simulink model "Buck_28V_12V_Analysis"  (R2023a)
settings: Solver=ode23t  StartTime=0.0  StopTime=0.05  MaxStep=1e-6  RelTol=1e-3
undefined symbols (not defined in the file): Rload
libraries: ee_lib x34, nesl_utility x33, fl_lib x26, simulink x24, slpidlib x4, simulink_extras x3
(part 1 of 2)
settings Model: Creator=MEHMET  LastModifiedBy=MEHMET

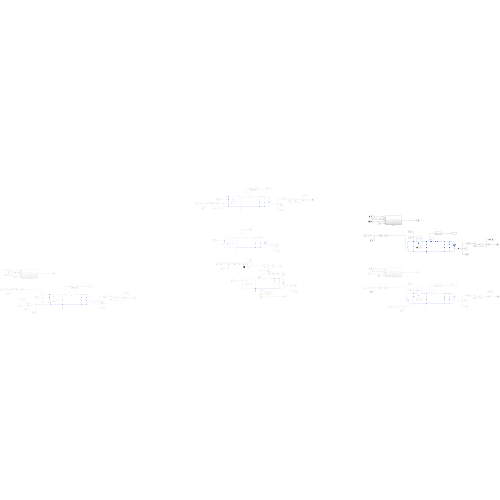
[thumbnail: Simulink's stored preview of the top-level diagram]
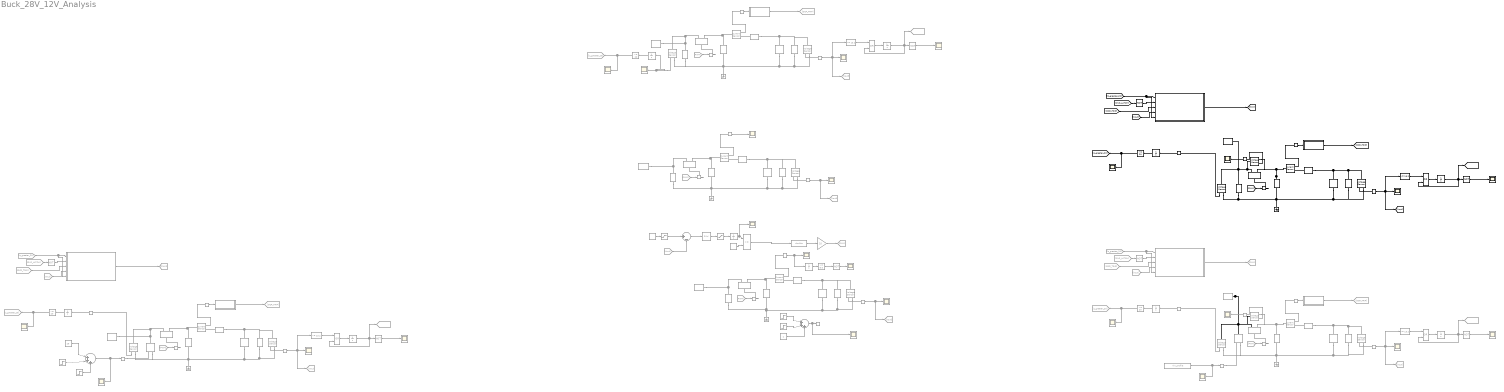
== system Buck_28V_12V_Analysis ==
  Capacitor{,1..3} (4 alike) : ee_lib/Passive/Capacitor  Commented=on  cap_option=ee.enum.passive.capacitor.capOption.const  c=220 uF  Cvec=[1e-05, 1e-06] F  Vvec=[0, 10] V  CV_table_symmetry=ee.enum.passive.capacitor.tableSymmetry.yes  f_vec=[1, 10] kHz  DFext_vec=[.8, 1.2]  enable_C_tol=ee.enum.toleranceApplication.none  averaging_period=0 s  C_tol=5  tol_distribution=ee.enum.toleranceDistribution.uniform  nSigma=4  r=1e-6 Ohm  g=0 1/Ohm  enable_operating_limits=ee.enum.enable.no  enable_faults=ee.enum.enable.no  fault_action=simscape.enum.assert.action.none  Cscale_faulted=100  R_faulted=1e-3 Ohm  G_faulted=0 1/Ohm  tau_fault=1e-3 s  fault_trigger=ee.enum.faults.faultTrigger.temporal  t_fault=1 s  max_permissible_voltage_range=[-100, 100] V  t_fail_on_voltage=1 s  operating_limit_action=ee.enum.passive.reportOpLim.warn  max_working_voltage_range=[-25, 25] V  power_rating=1 W  i_specify=off  i_priority=None  i=0 A  i_nominal_specify=off  i_nominal_unit=A  i_nominal_value=1  v_specify=off  v_priority=None  v=0 V  v_nominal_specify=off  v_nominal_unit=V  v_nominal_value=1  vc_specify=off  vc_priority=High  vc=0 V  vc_nominal_specify=off  vc_nominal_unit=V  vc_nominal_value=1
  Capacitor4 : ee_lib/Passive/Capacitor  cap_option=ee.enum.passive.capacitor.capOption.const  c=220 uF  Cvec=[1e-05, 1e-06] F  Vvec=[0, 10] V  CV_table_symmetry=ee.enum.passive.capacitor.tableSymmetry.yes  f_vec=[1, 10] kHz  DFext_vec=[.8, 1.2]  enable_C_tol=ee.enum.toleranceApplication.none  averaging_period=0 s  C_tol=5  tol_distribution=ee.enum.toleranceDistribution.uniform  nSigma=4  r=1e-6 Ohm  g=0 1/Ohm  enable_operating_limits=ee.enum.enable.no  enable_faults=ee.enum.enable.no  fault_action=simscape.enum.assert.action.none  Cscale_faulted=100  R_faulted=1e-3 Ohm  G_faulted=0 1/Ohm  tau_fault=1e-3 s  fault_trigger=ee.enum.faults.faultTrigger.temporal  t_fault=1 s  max_permissible_voltage_range=[-100, 100] V  t_fail_on_voltage=1 s  operating_limit_action=ee.enum.passive.reportOpLim.warn  max_working_voltage_range=[-25, 25] V  power_rating=1 W  i_specify=off  i_priority=None  i=0 A  i_nominal_specify=off  i_nominal_unit=A  i_nominal_value=1  v_specify=off  v_priority=None  v=0 V  v_nominal_specify=off  v_nominal_unit=V  v_nominal_value=1  vc_specify=off  vc_priority=High  vc=0 V  vc_nominal_specify=off  vc_nominal_unit=V  vc_nominal_value=1
  Capacitor5 : ee_lib/Passive/Capacitor  Commented=on  cap_option=ee.enum.passive.capacitor.capOption.const  c=C_test F  Cvec=[1e-05, 1e-06] F  Vvec=[0, 10] V  CV_table_symmetry=ee.enum.passive.capacitor.tableSymmetry.yes  f_vec=[1, 10] kHz  DFext_vec=[.8, 1.2]  enable_C_tol=ee.enum.toleranceApplication.none  averaging_period=0 s  C_tol=5  tol_distribution=ee.enum.toleranceDistribution.uniform  nSigma=4  r=ESR_test Ohm  g=0 1/Ohm  enable_operating_limits=ee.enum.enable.no  enable_faults=ee.enum.enable.no  fault_action=simscape.enum.assert.action.none  Cscale_faulted=100  R_faulted=1e-3 Ohm  G_faulted=0 1/Ohm  tau_fault=1e-3 s  fault_trigger=ee.enum.faults.faultTrigger.temporal  t_fault=1 s  max_permissible_voltage_range=[-100, 100] V  t_fail_on_voltage=1 s  operating_limit_action=ee.enum.passive.reportOpLim.warn  max_working_voltage_range=[-25, 25] V  power_rating=1 W  i_specify=off  i_priority=None  i=0 A  i_nominal_specify=off  i_nominal_unit=A  i_nominal_value=1  v_specify=off  v_priority=None  v=0 V  v_nominal_specify=off  v_nominal_unit=V  v_nominal_value=1  vc_specify=off  vc_priority=High  vc=0 V  vc_nominal_specify=off  vc_nominal_unit=V  vc_nominal_value=1
  Compare : Scope  Commented=on
  Compare To Constant : simulink/Logic and Bit Operations/Compare To Constant  Commented=on  relop=>=  const=6.0  OutDataTypeStr=boolean  ZeroCross=off
  Compare To Constant1 : simulink/Logic and Bit Operations/Compare To Constant  Commented=on  relop=>=  const=13.2  OutDataTypeStr=boolean  ZeroCross=off
  Compare To Constant2 : simulink/Logic and Bit Operations/Compare To Constant  Commented=on  relop=>=  const=20  OutDataTypeStr=boolean  ZeroCross=off
  Compare To Constant3 : simulink/Logic and Bit Operations/Compare To Constant  Commented=on  relop=>=  const=13.2  OutDataTypeStr=boolean  ZeroCross=off
  Compare To Constant4 : simulink/Logic and Bit Operations/Compare To Constant  Commented=on  relop=>=  const=20  OutDataTypeStr=boolean  ZeroCross=off
  Compare To Constant5 : simulink/Logic and Bit Operations/Compare To Constant  relop=>=  const=13.2  OutDataTypeStr=boolean  ZeroCross=off
  Compare To Constant6 : simulink/Logic and Bit Operations/Compare To Constant  relop=>=  const=20  OutDataTypeStr=boolean  ZeroCross=off
  Compare To Constant7 : simulink/Logic and Bit Operations/Compare To Constant  Commented=on  relop=>=  const=13.2  OutDataTypeStr=boolean  ZeroCross=off
  Compare To Constant8 : simulink/Logic and Bit Operations/Compare To Constant  Commented=on  relop=>=  const=20  OutDataTypeStr=boolean  ZeroCross=off
  Constant : Constant  Commented=on  Value=28
  Constant1 : Constant  Commented=on
  Controlled Voltage Source : fl_lib/Electrical/Electrical Sources/Controlled Voltage Source  Commented=on
  Controlled Voltage Source1 : fl_lib/Electrical/Electrical Sources/Controlled Voltage Source  Commented=on
  Current Sensor{,1..3,5} (5 alike) : fl_lib/Electrical/Electrical Sensors/Current Sensor  Commented=on
  Current Sensor4 : fl_lib/Electrical/Electrical Sensors/Current Sensor
  Current_Scope : Scope  Commented=on
  Current_Scope1 : Scope  Commented=on
  Current_is_greater_6A : Subsystem  Commented=on
  Current_is_greater_6A1 : Subsystem  Commented=on
  Current_is_greater_6A2 : Subsystem
  Current_is_greater_6A3 : Subsystem  Commented=on
  DC Voltage Source : ee_lib/Additional Components/SPICE Sources/DC Voltage Source  Commented=on  DC=28 V
  DC Voltage Source1 : ee_lib/Additional Components/SPICE Sources/DC Voltage Source  Commented=on  DC=Vin V
  DC Voltage Source2 : ee_lib/Additional Components/SPICE Sources/DC Voltage Source  Commented=on  DC=Vin V
  DC Voltage Source3 : ee_lib/Additional Components/SPICE Sources/DC Voltage Source  DC=28 V
  Data Type Conversion : DataTypeConversion  Commented=on  OutDataTypeStr=double  SaturateOnIntegerOverflow=off  RndMeth=Floor
  Diode{,1..3} (4 alike) : ee_lib/Semiconductors & Converters/Diode  Commented=on  ModelType=ee.enum.diode.modelType.pwl  TableType=ee.enum.diode.tableType.IfMat  IfMat=[.07, .12, .19, 1.75, 4.24, 7.32, 11.2; .16, .3, .72, 2.14, 5.02, 8.35, 13.12] A  VfMat=[.9, 1.15, 1.25, 1.5, 1.75, 2.17, 2.6, 2.85; .58, .68, .75, 1.1, 1.38, 1.77, 2.27, 2.7] V  TjVec=[25, 125] degC  VfVec=[.5, .7, .9, 1.3, 1.7, 2.1, 2.5] V  IfVec=[.1, .2, .5, 1, 2, 4, 7, 10] A  Vf=0.6 V  Ron=0.3 Ohm  Goff=1e-8 S  prmExp=ee.enum.diode.expParam.useTwo  I12=[.0137, .545] A  V12=[.6, .7] V  RS=0 Ohm  Tmeas=25 degC  IS=1e-12 A  ec=1  I1=0.0137 A  V1=0.6 V  N_series=1  N_parallel=1  Rz=0.3 Ohm  BV=inf V  C_param=ee.enum.diode.capParam.fixed  CJ=0 pF  CJ0=5 pF  Vvec=[.1, 10, 100] V  Cvec=[3.5, 1, .4] pF  VJ=1 V  Mgrad=0.5  FC=0.5  Q_param=ee.enum.diode.recoveryParam.off  iRM=-7.15 A  iF=4 A  didt=-750 A/us  trr_factor=3  trr=115 ns  Qrr=150 nA*s  Vr=-600 V  Ls=150 nH  Erec=0.03 J  TT=50 ns  tau=100 ns  T_param=ee.enum.diode.temperatureParam.off  Tdevice=25 degC  I1_T2=0.245 A  V1_T2=0.5 V  IS_T2=1.25e-7 A  Tmeas2=125 degC  XTI_param=ee.enum.diode.xtiParam.pn  XTI=3  EG_param=ee.enum.diode.egapParam.material_si  EG=1.11 eV  dBVdT=0 V/K  enable_faults=simscape.enum.onoff.off  fault_action=simscape.enum.assert.action.none  fault_types=ee.enum.diode.faults.open  tau_fault=1e-3 s  IfMat_faulted=[.07, .12, .19, 1.75, 4.24, 7.32, 11.2; .16, .3, .72, 2.14, 4.02, 6.35, 9.12] A  VfMat_faulted=[.9, 1.15, 1.25, 1.5, 1.75, 2.17, 2.6, 2.85; .58, .68, .75, 1.1, 1.38, 1.77, 2.27, 2.7] V  VfVec_faulted=[.5, .7, .9, 1.3, 1.7, 2.1, 2.5] V  IfVec_faulted=[.1, .2, .5, 1, 2, 4, 7, 10] A  Ropen_faulted=1000 Ohm  Gshort_faulted=1000 1/Ohm  Vf_faulted=0.6 V  Ron_faulted=0.3 Ohm  Goff_faulted=1e-8 S  I12_faulted=[.0137, .545] A  V12_faulted=[.6, .7] V  IS_faulted=1e-12 A  ec_faulted=1  I1_faulted=0.0137 A  V1_faulted=0.6 V  RS_faulted=0 Ohm  Rz_faulted=0.3 Ohm  BV_faulted=inf V  Cscale_faulted=100  fault_trigger=ee.enum.faults.faultTrigger.temporal  t_fault=inf s  max_permissible_voltage=inf V  n_fail_on_voltage=1  max_permissible_current=inf A  t_fail_on_current=1 s  max_permissible_dVdt=inf V/s  enable_fault_input=simscape.enum.onoff.off  i_specify=off  i_priority=None  i=0 A  i_nominal_specify=off  i_nominal_unit=A  i_nominal_value=1  v_specify=off  v_priority=None  v=0 V  v_nominal_specify=off  v_nominal_unit=V  v_nominal_value=1  v_capacitor_specify=off  v_capacitor_priority=None  v_capacitor=0 V  v_capacitor_nominal_specify=off  v_capacitor_nominal_unit=V  v_capacitor_nominal_value=1  i_diode_specify=off  i_diode_priority=None  i_diode=0 A  i_diode_nominal_specify=off  i_diode_nominal_unit=A  i_diode_nominal_value=1  v_diode_specify=off  v_diode_priority=None  v_diode=0 V  v_diode_nominal_specify=off  v_diode_nominal_unit=V  v_diode_nominal_value=1  i_capacitor_specify=off  i_capacitor_priority=None  i_capacitor=0 A  i_capacitor_nominal_specify=off  i_capacitor_nominal_unit=A  i_capacitor_nominal_value=1  power_dissipated_specify=off  power_dissipated_priority=None  power_dissipated=0 W  power_dissipated_nominal_specify=off  power_dissipated_nominal_unit=W  power_dissipated_nominal_value=1  fidelity_level=ee.enum.diode.fidelity.includeChargeDyn  rec_loss_model=ee.enum.diode.reverseRecoveryModel.fixed  ErecVal=0 J  ErecMat=zeros(2, 3) J  TjrecVec=[298.15, 398.15] K  IfrecVec=[.1, 1, 10] A  VrecVal=10 V  tFilter=1 / 1000 / 100 s  max_permissible_temperature=inf K  t_fail_on_temperature=1 s  thermal_network_parameterization=ee.enum.thermalNetworkTopology.junctionCase  Rth=[0, 10] K/W  Rth_Cauer=[1, 3, 10] K/W  Rth_Foster=[4, 6] K/W  thermal_mass_parameterization=ee.enum.thermalNetwork.timeconstant  thermal_mass=[0, 1] J/K  thermal_mass_Cauer=[.1, .3, 1] J/K  thermal_mass_Foster=[1.5, 3] J/K  thermal_time_constant=[0, 10] s  thermal_time_constant_Cauer=[1, 3, 10] s  thermal_time_constant_Foster=[6, 18] s  thermal_mass_initial_temperatures=[25, 25] degC  thermal_mass_initial_temperatures_Cauer=[25, 25, 25] degC  junction_thermal_mass=0.01 J/K  Tvec_initial_Foster=[25, 25, 25, 25] degC  no_thermal_network=0  junction_temperature_specify=off  junction_temperature_priority=None  junction_temperature=25 degC  junction_temperature_nominal_specify=off  junction_temperature_nominal_unit=degC  junction_temperature_nominal_value=1
  Diode4 : ee_lib/Semiconductors & Converters/Diode  ModelType=ee.enum.diode.modelType.pwl  TableType=ee.enum.diode.tableType.IfMat  IfMat=[.07, .12, .19, 1.75, 4.24, 7.32, 11.2; .16, .3, .72, 2.14, 5.02, 8.35, 13.12] A  VfMat=[.9, 1.15, 1.25, 1.5, 1.75, 2.17, 2.6, 2.85; .58, .68, .75, 1.1, 1.38, 1.77, 2.27, 2.7] V  TjVec=[25, 125] degC  VfVec=[.5, .7, .9, 1.3, 1.7, 2.1, 2.5] V  IfVec=[.1, .2, .5, 1, 2, 4, 7, 10] A  Vf=0.6 V  Ron=0.3 Ohm  Goff=1e-8 S  prmExp=ee.enum.diode.expParam.useTwo  I12=[.0137, .545] A  V12=[.6, .7] V  RS=0 Ohm  Tmeas=25 degC  IS=1e-12 A  ec=1  I1=0.0137 A  V1=0.6 V  N_series=1  N_parallel=1  Rz=0.3 Ohm  BV=inf V  C_param=ee.enum.diode.capParam.fixed  CJ=0 pF  CJ0=5 pF  Vvec=[.1, 10, 100] V  Cvec=[3.5, 1, .4] pF  VJ=1 V  Mgrad=0.5  FC=0.5  Q_param=ee.enum.diode.recoveryParam.off  iRM=-7.15 A  iF=4 A  didt=-750 A/us  trr_factor=3  trr=115 ns  Qrr=150 nA*s  Vr=-600 V  Ls=150 nH  Erec=0.03 J  TT=50 ns  tau=100 ns  T_param=ee.enum.diode.temperatureParam.off  Tdevice=25 degC  I1_T2=0.245 A  V1_T2=0.5 V  IS_T2=1.25e-7 A  Tmeas2=125 degC  XTI_param=ee.enum.diode.xtiParam.pn  XTI=3  EG_param=ee.enum.diode.egapParam.material_si  EG=1.11 eV  dBVdT=0 V/K  enable_faults=simscape.enum.onoff.off  fault_action=simscape.enum.assert.action.none  fault_types=ee.enum.diode.faults.open  tau_fault=1e-3 s  IfMat_faulted=[.07, .12, .19, 1.75, 4.24, 7.32, 11.2; .16, .3, .72, 2.14, 4.02, 6.35, 9.12] A  VfMat_faulted=[.9, 1.15, 1.25, 1.5, 1.75, 2.17, 2.6, 2.85; .58, .68, .75, 1.1, 1.38, 1.77, 2.27, 2.7] V  VfVec_faulted=[.5, .7, .9, 1.3, 1.7, 2.1, 2.5] V  IfVec_faulted=[.1, .2, .5, 1, 2, 4, 7, 10] A  Ropen_faulted=1000 Ohm  Gshort_faulted=1000 1/Ohm  Vf_faulted=0.6 V  Ron_faulted=0.3 Ohm  Goff_faulted=1e-8 S  I12_faulted=[.0137, .545] A  V12_faulted=[.6, .7] V  IS_faulted=1e-12 A  ec_faulted=1  I1_faulted=0.0137 A  V1_faulted=0.6 V  RS_faulted=0 Ohm  Rz_faulted=0.3 Ohm  BV_faulted=inf V  Cscale_faulted=100  fault_trigger=ee.enum.faults.faultTrigger.temporal  t_fault=inf s  max_permissible_voltage=inf V  n_fail_on_voltage=1  max_permissible_current=inf A  t_fail_on_current=1 s  max_permissible_dVdt=inf V/s  enable_fault_input=simscape.enum.onoff.off  i_specify=off  i_priority=None  i=0 A  i_nominal_specify=off  i_nominal_unit=A  i_nominal_value=1  v_specify=off  v_priority=None  v=0 V  v_nominal_specify=off  v_nominal_unit=V  v_nominal_value=1  v_capacitor_specify=off  v_capacitor_priority=None  v_capacitor=0 V  v_capacitor_nominal_specify=off  v_capacitor_nominal_unit=V  v_capacitor_nominal_value=1  i_diode_specify=off  i_diode_priority=None  i_diode=0 A  i_diode_nominal_specify=off  i_diode_nominal_unit=A  i_diode_nominal_value=1  v_diode_specify=off  v_diode_priority=None  v_diode=0 V  v_diode_nominal_specify=off  v_diode_nominal_unit=V  v_diode_nominal_value=1  i_capacitor_specify=off  i_capacitor_priority=None  i_capacitor=0 A  i_capacitor_nominal_specify=off  i_capacitor_nominal_unit=A  i_capacitor_nominal_value=1  power_dissipated_specify=off  power_dissipated_priority=None  power_dissipated=0 W  power_dissipated_nominal_specify=off  power_dissipated_nominal_unit=W  power_dissipated_nominal_value=1  fidelity_level=ee.enum.diode.fidelity.includeChargeDyn  rec_loss_model=ee.enum.diode.reverseRecoveryModel.fixed  ErecVal=0 J  ErecMat=zeros(2, 3) J  TjrecVec=[298.15, 398.15] K  IfrecVec=[.1, 1, 10] A  VrecVal=10 V  tFilter=1 / 1000 / 100 s  max_permissible_temperature=inf K  t_fail_on_temperature=1 s  thermal_network_parameterization=ee.enum.thermalNetworkTopology.junctionCase  Rth=[0, 10] K/W  Rth_Cauer=[1, 3, 10] K/W  Rth_Foster=[4, 6] K/W  thermal_mass_parameterization=ee.enum.thermalNetwork.timeconstant  thermal_mass=[0, 1] J/K  thermal_mass_Cauer=[.1, .3, 1] J/K  thermal_mass_Foster=[1.5, 3] J/K  thermal_time_constant=[0, 10] s  thermal_time_constant_Cauer=[1, 3, 10] s  thermal_time_constant_Foster=[6, 18] s  thermal_mass_initial_temperatures=[25, 25] degC  thermal_mass_initial_temperatures_Cauer=[25, 25, 25] degC  junction_thermal_mass=0.01 J/K  Tvec_initial_Foster=[25, 25, 25, 25] degC  no_thermal_network=0  junction_temperature_specify=off  junction_temperature_priority=None  junction_temperature=25 degC  junction_temperature_nominal_specify=off  junction_temperature_nominal_unit=degC  junction_temperature_nominal_value=1
  Diode5 : ee_lib/Semiconductors & Converters/Diode  Commented=on  ModelType=ee.enum.diode.modelType.pwl  TableType=ee.enum.diode.tableType.IfMat  IfMat=[.07, .12, .19, 1.75, 4.24, 7.32, 11.2; .16, .3, .72, 2.14, 5.02, 8.35, 13.12] A  VfMat=[.9, 1.15, 1.25, 1.5, 1.75, 2.17, 2.6, 2.85; .58, .68, .75, 1.1, 1.38, 1.77, 2.27, 2.7] V  TjVec=[25, 125] degC  VfVec=[.5, .7, .9, 1.3, 1.7, 2.1, 2.5] V  IfVec=[.1, .2, .5, 1, 2, 4, 7, 10] A  Vf=0.6 V  Ron=0.01 Ohm  Goff=1e-8 S  prmExp=ee.enum.diode.expParam.useTwo  I12=[.0137, .545] A  V12=[.6, .7] V  RS=0 Ohm  Tmeas=25 degC  IS=1e-12 A  ec=1  I1=0.0137 A  V1=0.6 V  N_series=1  N_parallel=1  Rz=0.3 Ohm  BV=inf V  C_param=ee.enum.diode.capParam.fixed  CJ=0 pF  CJ0=5 pF  Vvec=[.1, 10, 100] V  Cvec=[3.5, 1, .4] pF  VJ=1 V  Mgrad=0.5  FC=0.5  Q_param=ee.enum.diode.recoveryParam.off  iRM=-7.15 A  iF=4 A  didt=-750 A/us  trr_factor=3  trr=115 ns  Qrr=150 nA*s  Vr=-600 V  Ls=150 nH  Erec=0.03 J  TT=50 ns  tau=100 ns  T_param=ee.enum.diode.temperatureParam.off  Tdevice=25 degC  I1_T2=0.245 A  V1_T2=0.5 V  IS_T2=1.25e-7 A  Tmeas2=125 degC  XTI_param=ee.enum.diode.xtiParam.pn  XTI=3  EG_param=ee.enum.diode.egapParam.material_si  EG=1.11 eV  dBVdT=0 V/K  enable_faults=simscape.enum.onoff.off  fault_action=simscape.enum.assert.action.none  fault_types=ee.enum.diode.faults.open  tau_fault=1e-3 s  IfMat_faulted=[.07, .12, .19, 1.75, 4.24, 7.32, 11.2; .16, .3, .72, 2.14, 4.02, 6.35, 9.12] A  VfMat_faulted=[.9, 1.15, 1.25, 1.5, 1.75, 2.17, 2.6, 2.85; .58, .68, .75, 1.1, 1.38, 1.77, 2.27, 2.7] V  VfVec_faulted=[.5, .7, .9, 1.3, 1.7, 2.1, 2.5] V  IfVec_faulted=[.1, .2, .5, 1, 2, 4, 7, 10] A  Ropen_faulted=1000 Ohm  Gshort_faulted=1000 1/Ohm  Vf_faulted=0.6 V  Ron_faulted=0.3 Ohm  Goff_faulted=1e-8 S  I12_faulted=[.0137, .545] A  V12_faulted=[.6, .7] V  IS_faulted=1e-12 A  ec_faulted=1  I1_faulted=0.0137 A  V1_faulted=0.6 V  RS_faulted=0 Ohm  Rz_faulted=0.3 Ohm  BV_faulted=inf V  Cscale_faulted=100  fault_trigger=ee.enum.faults.faultTrigger.temporal  t_fault=inf s  max_permissible_voltage=inf V  n_fail_on_voltage=1  max_permissible_current=inf A  t_fail_on_current=1 s  max_permissible_dVdt=inf V/s  enable_fault_input=simscape.enum.onoff.off  i_specify=off  i_priority=None  i=0 A  i_nominal_specify=off  i_nominal_unit=A  i_nominal_value=1  v_specify=off  v_priority=None  v=0 V  v_nominal_specify=off  v_nominal_unit=V  v_nominal_value=1  v_capacitor_specify=off  v_capacitor_priority=None  v_capacitor=0 V  v_capacitor_nominal_specify=off  v_capacitor_nominal_unit=V  v_capacitor_nominal_value=1  i_diode_specify=off  i_diode_priority=None  i_diode=0 A  i_diode_nominal_specify=off  i_diode_nominal_unit=A  i_diode_nominal_value=1  v_diode_specify=off  v_diode_priority=None  v_diode=0 V  v_diode_nominal_specify=off  v_diode_nominal_unit=V  v_diode_nominal_value=1  i_capacitor_specify=off  i_capacitor_priority=None  i_capacitor=0 A  i_capacitor_nominal_specify=off  i_capacitor_nominal_unit=A  i_capacitor_nominal_value=1  power_dissipated_specify=off  power_dissipated_priority=None  power_dissipated=0 W  power_dissipated_nominal_specify=off  power_dissipated_nominal_unit=W  power_dissipated_nominal_value=1  fidelity_level=ee.enum.diode.fidelity.includeChargeDyn  rec_loss_model=ee.enum.diode.reverseRecoveryModel.fixed  ErecVal=0 J  ErecMat=zeros(2, 3) J  TjrecVec=[298.15, 398.15] K  IfrecVec=[.1, 1, 10] A  VrecVal=10 V  tFilter=1 / 1000 / 100 s  max_permissible_temperature=inf K  t_fail_on_temperature=1 s  thermal_network_parameterization=ee.enum.thermalNetworkTopology.junctionCase  Rth=[0, 10] K/W  Rth_Cauer=[1, 3, 10] K/W  Rth_Foster=[4, 6] K/W  thermal_mass_parameterization=ee.enum.thermalNetwork.timeconstant  thermal_mass=[0, 1] J/K  thermal_mass_Cauer=[.1, .3, 1] J/K  thermal_mass_Foster=[1.5, 3] J/K  thermal_time_constant=[0, 10] s  thermal_time_constant_Cauer=[1, 3, 10] s  thermal_time_constant_Foster=[6, 18] s  thermal_mass_initial_temperatures=[25, 25] degC  thermal_mass_initial_temperatures_Cauer=[25, 25, 25] degC  junction_thermal_mass=0.01 J/K  Tvec_initial_Foster=[25, 25, 25, 25] degC  no_thermal_network=0  junction_temperature_specify=off  junction_temperature_priority=None  junction_temperature=25 degC  junction_temperature_nominal_specify=off  junction_temperature_nominal_unit=degC  junction_temperature_nominal_value=1
  Electrical Reference{,1..3,5} (5 alike) : fl_lib/Electrical/Electrical Elements/Electrical Reference  Commented=on
  Electrical Reference4 : fl_lib/Electrical/Electrical Elements/Electrical Reference
  From : From  Commented=on  GotoTag=Vout
  From Workspace : FromWorkspace  Commented=on  VariableName=Vin_profile  Interpolate=off  ZeroCross=off  OutputAfterFinalValue=Holding final value
  From{1..2,4,8,17} (5 alike) : From  Commented=on  GotoTag=PWM
  From14 : From  Commented=on  GotoTag=OCP_TRIP
  From15 : From  Commented=on  GotoTag=OVP_LATCH
  From16 : From  Commented=on  GotoTag=is_greater_20
  From18 : From  Commented=on  GotoTag=Vout
  From3 : From  Commented=on  GotoTag=Vout
  From5 : From  Commented=on  GotoTag=OCP_TRIP
  From6 : From  Commented=on  GotoTag=OVP_LATCH
  From7 : From  Commented=on  GotoTag=is_greater_20
  Gain : Gain  Commented=on  Gain=10
  Goto{,2..3,8,20} (5 alike) : Goto  Commented=on  GotoTag=Vout
  Goto1 : Goto  Commented=on  GotoTag=PWM
  Goto10 : Goto  Commented=on  GotoTag=OVP_LATCH
  Goto11 : Goto  Commented=on  GotoTag=is_greater_20
  Goto17 : Goto  Commented=on  GotoTag=OVP_LATCH
  Goto18 : Goto  Commented=on  GotoTag=is_greater_20
  Goto19 : Goto  Commented=on  GotoTag=PWM
  Goto21 : Goto  Commented=on  GotoTag=OCP_TRIP
  Goto4 : Goto  Commented=on  GotoTag=PWM
  Goto5 : Goto  Commented=on  GotoTag=OCP_TRIP
  Goto6 : Goto  Commented=on  GotoTag=OVP_LATCH
  Goto7 : Goto  Commented=on  GotoTag=is_greater_20
  Goto9 : Goto  Commented=on  GotoTag=OCP_TRIP
  Inductor{,1..3} (4 alike) : ee_lib/Passive/Inductor  Commented=on  l=47 uH  enable_L_tol=ee.enum.toleranceApplication.none  L_tol=20  tol_distribution=ee.enum.toleranceDistribution.uniform  nSigma=4  r=0 Ohm  g=1e-9 1/Ohm  enable_operating_limits=ee.enum.enable.no  operating_limit_action=ee.enum.passive.reportOpLim.warn  max_working_current=1 A  power_rating=1 W  enable_faults=ee.enum.enable.no  fault_action=simscape.enum.assert.action.none  lambdaPercent=50  k_faulted=0.9999  turnsShort=ee.enum.passive.inductor.turnsShortOption.no  openCct=ee.enum.enable.no  groundShort=ee.enum.passive.inductor.groundShortOption.no  groundShortG=0 1/Ohm  tau_fault=1e-3 s  fault_trigger=ee.enum.faults.faultTrigger.temporal  t_fault=1 s  max_permissible_voltage=100 V  n_fail_on_voltage=1  max_permissible_current=1 A  t_fail_on_current=1 s  i_L_specify=off  i_L_priority=High  i_L=0 A  i_L_nominal_specify=off  i_L_nominal_unit=A  i_L_nominal_value=1
  Inductor4 : ee_lib/Passive/Inductor  l=47 uH  enable_L_tol=ee.enum.toleranceApplication.none  L_tol=20  tol_distribution=ee.enum.toleranceDistribution.uniform  nSigma=4  r=0 Ohm  g=1e-9 1/Ohm  enable_operating_limits=ee.enum.enable.no  operating_limit_action=ee.enum.passive.reportOpLim.warn  max_working_current=1 A  power_rating=1 W  enable_faults=ee.enum.enable.no  fault_action=simscape.enum.assert.action.none  lambdaPercent=50  k_faulted=0.9999  turnsShort=ee.enum.passive.inductor.turnsShortOption.no  openCct=ee.enum.enable.no  groundShort=ee.enum.passive.inductor.groundShortOption.no  groundShortG=0 1/Ohm  tau_fault=1e-3 s  fault_trigger=ee.enum.faults.faultTrigger.temporal  t_fault=1 s  max_permissible_voltage=100 V  n_fail_on_voltage=1  max_permissible_current=1 A  t_fail_on_current=1 s  i_L_specify=off  i_L_priority=High  i_L=0 A  i_L_nominal_specify=off  i_L_nominal_unit=A  i_L_nominal_value=1
  Inductor5 : ee_lib/Passive/Inductor  Commented=on  l=L_test H  enable_L_tol=ee.enum.toleranceApplication.none  L_tol=20  tol_distribution=ee.enum.toleranceDistribution.uniform  nSigma=4  r=RL_test Ohm  g=1e-9 1/Ohm  enable_operating_limits=ee.enum.enable.no  operating_limit_action=ee.enum.passive.reportOpLim.warn  max_working_current=1 A  power_rating=1 W  enable_faults=ee.enum.enable.no  fault_action=simscape.enum.assert.action.none  lambdaPercent=50  k_faulted=0.9999  turnsShort=ee.enum.passive.inductor.turnsShortOption.no  openCct=ee.enum.enable.no  groundShort=ee.enum.passive.inductor.groundShortOption.no  groundShortG=0 1/Ohm  tau_fault=1e-3 s  fault_trigger=ee.enum.faults.faultTrigger.temporal  t_fault=1 s  max_permissible_voltage=100 V  n_fail_on_voltage=1  max_permissible_current=1 A  t_fail_on_current=1 s  i_L_specify=off  i_L_priority=High  i_L=0 A  i_L_nominal_specify=off  i_L_nominal_unit=A  i_L_nominal_value=1
  MOSFET (Ideal, Switching){,1..3,5} (5 alike) : ee_lib/Semiconductors & Converters/MOSFET (Ideal, Switching)  Commented=on  port_option=ee.enum.controlport.ps  Rds=0.01 Ohm  Goff=1e-6 1/Ohm  Vth=2 V  diode_param=ee.enum.converters.protectiondiode.none  diode_Vf=0.8 V  diode_Ron=0.001 Ohm  diode_Goff=1e-5 1/Ohm  diode_C=50e-9 F  diode_iRM=-235 A  diode_iF=300 A  diode_idot=-50 A/us  diode_trr_param=ee.enum.converters.diodeReverseParam.trr_factor  diode_trr_factor=3  diode_trr=15 us  diode_Qrr=1500 s*uA  ids_specify=off  ids_priority=None  ids=0 A  ids_nominal_specify=off  ids_nominal_unit=A  ids_nominal_value=1  vds_specify=off  vds_priority=None  vds=0 V  vds_nominal_specify=off  vds_nominal_unit=V  vds_nominal_value=1  vgs_specify=off  vgs_priority=None  vgs=0 V  vgs_nominal_specify=off  vgs_nominal_unit=V  vgs_nominal_value=1  thermal_loss_option=ee.enum.converters.thermalLossOption.constantvalues  Von_data=[0, 1.8, 3.2, 6, 10, 16; 0, 2, 5.5, 9.5, 15, 25] V  Tj=[298.15, 448.15] K  Iout_data=[0, 20, 40, 60, 80, 100] A  Eon_data=[0, 55.04, 124.57, 235.53, 362.12; 0, 71.25, 161.25, 304.88, 468.75] * 1e-6 J  Eoff_data=[0, 18, 30, 56.1, 76.5; 0, 22.5, 37.5, 70.13, 95.63] * 1e-6 J  Tj_loss=[298.15, 448.15] K  Iout_data_loss=[0, 10, 20, 30, 40] A  Eon_scalar=22.86e-3 J  Eoff_scalar=17.14e-3 J  Voff=300 V  Iout_scalar=600 A  diodeModelType=ee.enum.converters.diodeModelType.pwl  diodeTableType=ee.enum.diode.tableType.IfMat  diode_IfMat=[.07, .12, .19, 1.75, 4.24, 7.32, 11.2; .16, .3, .72, 2.14, 4.02, 6.35, 9.12] A  diode_VfMat=[.9, 1.15, 1.25, 1.5, 1.75, 2.17, 2.6, 2.85; .58, .68, .75, 1.1, 1.38, 1.77, 2.27, 2.7] V  diode_TjVec=[25, 125] degC  diode_VfVec=[.5, .7, .9, 1.3, 1.7, 2.1, 2.5] V  diode_IfVec=[.1, .2, .5, 1, 2, 4, 7, 10] A  diode_Vr=-600 V  diode_Ls=150 nH  diode_Erec=0.03 J  diode_rec_loss_model=ee.enum.diode.reverseRecoveryModel.fixed  diode_ErecVal=0 J  diode_ErecMat=zeros(2, 3) J  diode_TjrecVec=[298.15, 398.15] K  diode_IfrecVec=[.1, 1, 10] A  diode_VrecVal=10 V  diode_tFilter=1 / 1000 / 100 s  thermal_network_parameterization=ee.enum.thermalNetworkTopology.external  Rth=[.03, .2] K/W  Rth_Cauer=[.03, .1, .2] K/W  Rth_Foster=[.03, .2] K/W  thermal_mass_parameterization=ee.enum.thermalNetwork.timeconstant  thermal_mass=[3, 25] J/K  thermal_mass_Cauer=[3, 10, 25] J/K  thermal_mass_Foster=[33, 50] J/K  thermal_time_constant=[.1, 5] s  thermal_time_constant_Cauer=[.1, 1, 5] s  thermal_time_constant_Foster=[1, 10] s  thermal_mass_initial_temperatures=[25, 25] degC  thermal_mass_initial_temperatures_Cauer=[25, 25, 25] degC  junction_thermal_mass=0.1 J/K  Tvec_initial_Foster=[25, 25, 25, 25] degC  no_thermal_network=0  junction_temperature_specify=off  junction_temperature_priority=None  junction_temperature=25 degC  junction_temperature_nominal_specify=off  junction_temperature_nominal_unit=degC  junction_temperature_nominal_value=1  Qj_specify=off  Qj_priority=None  Qj=0 W  Qj_nominal_specify=off  Qj_nominal_unit=W  Qj_nominal_value=1
  "MOSFET (Ideal, Switching)4" : ee_lib/Semiconductors & Converters/MOSFET (Ideal, Switching)  port_option=ee.enum.controlport.ps  Rds=0.01 Ohm  Goff=1e-6 1/Ohm  Vth=2 V  diode_param=ee.enum.converters.protectiondiode.none  diode_Vf=0.8 V  diode_Ron=0.001 Ohm  diode_Goff=1e-5 1/Ohm  diode_C=50e-9 F  diode_iRM=-235 A  diode_iF=300 A  diode_idot=-50 A/us  diode_trr_param=ee.enum.converters.diodeReverseParam.trr_factor  diode_trr_factor=3  diode_trr=15 us  diode_Qrr=1500 s*uA  ids_specify=off  ids_priority=None  ids=0 A  ids_nominal_specify=off  ids_nominal_unit=A  ids_nominal_value=1  vds_specify=off  vds_priority=None  vds=0 V  vds_nominal_specify=off  vds_nominal_unit=V  vds_nominal_value=1  vgs_specify=off  vgs_priority=None  vgs=0 V  vgs_nominal_specify=off  vgs_nominal_unit=V  vgs_nominal_value=1  thermal_loss_option=ee.enum.converters.thermalLossOption.constantvalues  Von_data=[0, 1.8, 3.2, 6, 10, 16; 0, 2, 5.5, 9.5, 15, 25] V  Tj=[298.15, 448.15] K  Iout_data=[0, 20, 40, 60, 80, 100] A  Eon_data=[0, 55.04, 124.57, 235.53, 362.12; 0, 71.25, 161.25, 304.88, 468.75] * 1e-6 J  Eoff_data=[0, 18, 30, 56.1, 76.5; 0, 22.5, 37.5, 70.13, 95.63] * 1e-6 J  Tj_loss=[298.15, 448.15] K  Iout_data_loss=[0, 10, 20, 30, 40] A  Eon_scalar=22.86e-3 J  Eoff_scalar=17.14e-3 J  Voff=300 V  Iout_scalar=600 A  diodeModelType=ee.enum.converters.diodeModelType.pwl  diodeTableType=ee.enum.diode.tableType.IfMat  diode_IfMat=[.07, .12, .19, 1.75, 4.24, 7.32, 11.2; .16, .3, .72, 2.14, 4.02, 6.35, 9.12] A  diode_VfMat=[.9, 1.15, 1.25, 1.5, 1.75, 2.17, 2.6, 2.85; .58, .68, .75, 1.1, 1.38, 1.77, 2.27, 2.7] V  diode_TjVec=[25, 125] degC  diode_VfVec=[.5, .7, .9, 1.3, 1.7, 2.1, 2.5] V  diode_IfVec=[.1, .2, .5, 1, 2, 4, 7, 10] A  diode_Vr=-600 V  diode_Ls=150 nH  diode_Erec=0.03 J  diode_rec_loss_model=ee.enum.diode.reverseRecoveryModel.fixed  diode_ErecVal=0 J  diode_ErecMat=zeros(2, 3) J  diode_TjrecVec=[298.15, 398.15] K  diode_IfrecVec=[.1, 1, 10] A  diode_VrecVal=10 V  diode_tFilter=1 / 1000 / 100 s  thermal_network_parameterization=ee.enum.thermalNetworkTopology.external  Rth=[.03, .2] K/W  Rth_Cauer=[.03, .1, .2] K/W  Rth_Foster=[.03, .2] K/W  thermal_mass_parameterization=ee.enum.thermalNetwork.timeconstant  thermal_mass=[3, 25] J/K  thermal_mass_Cauer=[3, 10, 25] J/K  thermal_mass_Foster=[33, 50] J/K  thermal_time_constant=[.1, 5] s  thermal_time_constant_Cauer=[.1, 1, 5] s  thermal_time_constant_Foster=[1, 10] s  thermal_mass_initial_temperatures=[25, 25] degC  thermal_mass_initial_temperatures_Cauer=[25, 25, 25] degC  junction_thermal_mass=0.1 J/K  Tvec_initial_Foster=[25, 25, 25, 25] degC  no_thermal_network=0  junction_temperature_specify=off  junction_temperature_priority=None  junction_temperature=25 degC  junction_temperature_nominal_specify=off  junction_temperature_nominal_unit=degC  junction_temperature_nominal_value=1  Qj_specify=off  Qj_priority=None  Qj=0 W  Qj_nominal_specify=off  Qj_nominal_unit=W  Qj_nominal_value=1
  NOT{,1..3,6..7} (6 alike) : Logic  Commented=on  Operator=NOT  IconShape=distinctive  AllPortsSameDT=off  OutDataTypeStr=boolean
  NOT4 : Logic  Operator=NOT  IconShape=distinctive  AllPortsSameDT=off  OutDataTypeStr=boolean
  NOT5 : Logic  Operator=NOT  IconShape=distinctive  AllPortsSameDT=off  OutDataTypeStr=boolean
  OR : Logic  Commented=on  Operator=OR  IconShape=distinctive  AllPortsSameDT=off  OutDataTypeStr=boolean
  OR1 : Logic  Commented=on  Operator=OR  IconShape=distinctive  AllPortsSameDT=off  OutDataTypeStr=boolean
  OR2 : Logic  Operator=OR  IconShape=distinctive  AllPortsSameDT=off  OutDataTypeStr=boolean
  OR3 : Logic  Commented=on  Operator=OR  IconShape=distinctive  AllPortsSameDT=off  OutDataTypeStr=boolean
  PID Controller : slpidlib/PID Controller  Commented=on  Controller=PI  Form=Parallel  TimeDomain=Continuous-time  UseExternalTs=off  SampleTime=-1  IntegratorMethod=Forward Euler  FilterMethod=Forward Euler  ControllerParametersSource=internal  P=0.02  I=50  UseKiTs=off  D=0  N=100  UseFilter=on  TunerSelectOption=Transfer Function Based (PID Tuner App)  ZeroCross=off  InitialConditionSource=internal  InitialConditionForIntegrator=0  InitialConditionForFilter=0  DifferentiatorICPrevScaledInput=0  ExternalReset=none  TrackingMode=off  Kt=1  LimitOutput=off  SatLimitsSource=internal  UpperSaturationLimit=inf  LowerSaturationLimit=-inf  LinearizeAsGain=on  AntiWindupMode=none  Kb=1  LimitIntegrator=off  UpperIntegratorSaturationLimit=inf  LowerIntegratorSaturationLimit=-inf  POutMin=[]  POutMax=[]  IOutMin=[]  IOutMax=[]  DOutMin=[]  DOutMax=[]  NOutMin=[]  NOutMax=[]  SumOutMin=[]  SumOutMax=[]  SaturationOutMin=[]  SaturationOutMax=[]  PParamMin=[]  PParamMax=[]  IParamMin=[]  IParamMax=[]  DParamMin=[]  DParamMax=[]  NParamMin=[]  NParamMax=[]  KbParamMin=[]  KbParamMax=[]  KtParamMin=[]  KtParamMax=[]  KbOutMin=[]  KbOutMax=[]  KtOutMin=[]  KtOutMax=[]  IntegratorOutMin=[]  IntegratorOutMax=[]  FilterOutMin=[]  FilterOutMax=[]  SumI1OutMin=[]  SumI1OutMax=[]  SumI2OutMin=[]  SumI2OutMax=[]  SumI3OutMin=[]  SumI3OutMax=[]  SumI4OutMin=[]  SumI4OutMax=[]  SumDOutMin=[]  SumDOutMax=[]  DifferentiatorOutMin=[]  DifferentiatorOutMax=[]  FilterDiffOutCoefMin=[]  FilterDiffOutCoefMax=[]  ReciprocalOutMin=[]  ReciprocalOutMax=[]  SumDenOutMin=[]  SumDenOutMax=[]  SumNumOutMin=[]  SumNumOutMax=[]  DivideOutMin=[]  DivideOutMax=[]  UdiffTsProdOutMin=[]  UdiffTsProdOutMax=[]  NTsProdOutMin=[]  NTsProdOutMax=[]  UintegralTsProdOutMin=[]  UintegralTsProdOutMax=[]  UngainTsProdOutMin=[]  UngainTsProdOutMax=[]  ClampingZeroOutDataTypeStr=Inherit: Inherit via back propagation  ClampingZeroOutMin=[]  ClampingZeroOutMax=[]  FilterDenConstantOutDataTypeStr=Inherit: Inherit via back propagation  FilterDenConstantOutMin=[]  FilterDenConstantOutMax=[]  PCopyOutDataTypeStr=Inherit: Inherit via back propagation  PCopyOutMin=[]  PCopyOutMax=[]  NCopyOutDataTypeStr=Inherit: Inherit via back propagation  NCopyOutMin=[]  NCopyOutMax=[]  IntegratorContinuousStateAttributes=''  IntegratorStateMustResolveToSignalObject=off  IntegratorRTWStateStorageClass=Auto  FilterContinuousStateAttributes=''  FilterStateMustResolveToSignalObject=off  FilterRTWStateStorageClass=Auto  ParallelPVariant=InternalParameters  IdealPVariant=Disabled  IVariant=InternalParameters  DVariant=Disabled  IntegratorVariant=Continuous  SatVariant=Disabled  AWVariant=Passthrough  PCopyVariant=Disabled  TRVariant=Disabled  FdbkBlocksVariant=Forward  IdealPFdbkVariant=Disabled  SatFdbkVariant=Disabled  DerivativeFilterVariant=Disabled  NVariant=Disabled  NCopyVariant=Disabled_SignalSpec  FilterICVariant=Disabled  IntegratorICVariant=InternalICs  ExternalResetVariant=Disabled  TRSumVariant=Passthrough  SumFdbkVariant=Disabled  SumVariant=Sum_PI  TsampFilterVariant=InternalTs  TsampNgainVariant=Passthrough  TsampIntegralVariant=Disabled_SignalSpec  ExternalSaturationOutDataTypeStr=Inherit: Same as second input
  PS-Simulink Converter{,1..9,14..17} (14 alike) : nesl_utility/PS-Simulink Converter  Commented=on  PhysicalDomain=network_engine_domain  SubClassName=ps_output  LeftPortType=input  RightPortType=output  PseudoPeriodic=off  Frequencies=[]  VectorFormat=inherit  Unit=inherit  AffineConversion=off
  PS-Simulink Converter{10..13} (4 alike) : nesl_utility/PS-Simulink Converter  PhysicalDomain=network_engine_domain  SubClassName=ps_output  LeftPortType=input  RightPortType=output  PseudoPeriodic=off  Frequencies=[]  VectorFormat=inherit  Unit=inherit  AffineConversion=off
  PWM : Subsystem  Commented=on
  PWM1 : Subsystem
  PWM2 : Subsystem  Commented=on
  Ramp : simulink/Sources/Ramp  Commented=on  slope=6000  start=0  InitialOutput=0
  Relational Operator : RelationalOperator  Commented=on  OutDataTypeStr=boolean  RndMeth=Simplest  InputSameDT=off
  Repeating Sequence : simulink/Sources/Repeating Sequence  Commented=on  rep_seq_t=[0 10e-6]  rep_seq_y=[0 1]
  Resistor : ee_lib/Passive/Resistor  Commented=on  R=2.4 Ohm  enable_R_tol=ee.enum.toleranceApplication.none  R_tol=5  tol_distribution=ee.enum.toleranceDistribution.uniform  nSigma=4  enable_operating_limits=ee.enum.enable.no  operating_limit_action=ee.enum.passive.reportOpLim.warn  power_rating=1 W  max_working_voltage=100 V  enable_faults=ee.enum.enable.no  fault_action=simscape.enum.assert.action.none  R_faulted=inf Ohm  fault_trigger=ee.enum.faults.faultTrigger.temporal  t_fault=1 s  max_permissible_current=1 A  t_fail_on_current=1 s  noise_mode=ee.enum.sources.noise.Disabled  Tdevice=25 degC  sample_time=1e-3 s  repeatability=ee.enum.ic.repeatability.notRepeatable  user_seed=0  auto_seed=3499211588  power_derating_T1=70 degC  power_derating_T2=155 degC  operating_temperature_range_vec=[-50, 150] degC  alpha=3.93e-3 1/K  Tmeas=25 degC  thermal_mass=100 J/K  temperature_specify=off  temperature_priority=High  temperature=298.15 K  temperature_nominal_specify=off  temperature_nominal_unit=K  temperature_nominal_value=1
  Resistor1 : ee_lib/Passive/Resistor  Commented=on  R=Rload Ohm  enable_R_tol=ee.enum.toleranceApplication.none  R_tol=5  tol_distribution=ee.enum.toleranceDistribution.uniform  nSigma=4  enable_operating_limits=ee.enum.enable.no  operating_limit_action=ee.enum.passive.reportOpLim.warn  power_rating=1 W  max_working_voltage=100 V  enable_faults=ee.enum.enable.no  fault_action=simscape.enum.assert.action.none  R_faulted=inf Ohm  fault_trigger=ee.enum.faults.faultTrigger.temporal  t_fault=1 s  max_permissible_current=1 A  t_fail_on_current=1 s  noise_mode=ee.enum.sources.noise.Disabled  Tdevice=25 degC  sample_time=1e-3 s  repeatability=ee.enum.ic.repeatability.notRepeatable  user_seed=0  auto_seed=3890346746  power_derating_T1=70 degC  power_derating_T2=155 degC  operating_temperature_range_vec=[-50, 150] degC  alpha=3.93e-3 1/K  Tmeas=25 degC  thermal_mass=100 J/K  temperature_specify=off  temperature_priority=High  temperature=298.15 K  temperature_nominal_specify=off  temperature_nominal_unit=K  temperature_nominal_value=1
  Resistor2 : ee_lib/Passive/Resistor  Commented=on  R=Rload Ohm  enable_R_tol=ee.enum.toleranceApplication.none  R_tol=5  tol_distribution=ee.enum.toleranceDistribution.uniform  nSigma=4  enable_operating_limits=ee.enum.enable.no  operating_limit_action=ee.enum.passive.reportOpLim.warn  power_rating=1 W  max_working_voltage=100 V  enable_faults=ee.enum.enable.no  fault_action=simscape.enum.assert.action.none  R_faulted=inf Ohm  fault_trigger=ee.enum.faults.faultTrigger.temporal  t_fault=1 s  max_permissible_current=1 A  t_fail_on_current=1 s  noise_mode=ee.enum.sources.noise.Disabled  Tdevice=25 degC  sample_time=1e-3 s  repeatability=ee.enum.ic.repeatability.notRepeatable  user_seed=0  auto_seed=3499211588  power_derating_T1=70 degC  power_derating_T2=155 degC  operating_temperature_range_vec=[-50, 150] degC  alpha=3.93e-3 1/K  Tmeas=25 degC  thermal_mass=100 J/K  temperature_specify=off  temperature_priority=High  temperature=298.15 K  temperature_nominal_specify=off  temperature_nominal_unit=K  temperature_nominal_value=1
  Resistor3 : ee_lib/Passive/Resistor  Commented=on  R=2.4 Ohm  enable_R_tol=ee.enum.toleranceApplication.none  R_tol=5  tol_distribution=ee.enum.toleranceDistribution.uniform  nSigma=4  enable_operating_limits=ee.enum.enable.no  operating_limit_action=ee.enum.passive.reportOpLim.warn  power_rating=1 W  max_working_voltage=100 V  enable_faults=ee.enum.enable.no  fault_action=simscape.enum.assert.action.none  R_faulted=inf Ohm  fault_trigger=ee.enum.faults.faultTrigger.temporal  t_fault=1 s  max_permissible_current=1 A  t_fail_on_current=1 s  noise_mode=ee.enum.sources.noise.Disabled  Tdevice=25 degC  sample_time=1e-3 s  repeatability=ee.enum.ic.repeatability.notRepeatable  user_seed=0  auto_seed=3499211588  power_derating_T1=70 degC  power_derating_T2=155 degC  operating_temperature_range_vec=[-50, 150] degC  alpha=3.93e-3 1/K  Tmeas=25 degC  thermal_mass=100 J/K  temperature_specify=off  temperature_priority=High  temperature=298.15 K  temperature_nominal_specify=off  temperature_nominal_unit=K  temperature_nominal_value=1
  Resistor4 : ee_lib/Passive/Resistor  R=2.4 Ohm  enable_R_tol=ee.enum.toleranceApplication.none  R_tol=5  tol_distribution=ee.enum.toleranceDistribution.uniform  nSigma=4  enable_operating_limits=ee.enum.enable.no  operating_limit_action=ee.enum.passive.reportOpLim.warn  power_rating=1 W  max_working_voltage=100 V  enable_faults=ee.enum.enable.no  fault_action=simscape.enum.assert.action.none  R_faulted=inf Ohm  fault_trigger=ee.enum.faults.faultTrigger.temporal  t_fault=1 s  max_permissible_current=1 A  t_fail_on_current=1 s  noise_mode=ee.enum.sources.noise.Disabled  Tdevice=25 degC  sample_time=1e-3 s  repeatability=ee.enum.ic.repeatability.notRepeatable  user_seed=0  auto_seed=3499211588  power_derating_T1=70 degC  power_derating_T2=155 degC  operating_temperature_range_vec=[-50, 150] degC  alpha=3.93e-3 1/K  Tmeas=25 degC  thermal_mass=100 J/K  temperature_specify=off  temperature_priority=High  temperature=298.15 K  temperature_nominal_specify=off  temperature_nominal_unit=K  temperature_nominal_value=1
  Resistor5 : ee_lib/Passive/Resistor  Commented=on  R=2.4 Ohm  enable_R_tol=ee.enum.toleranceApplication.none  R_tol=5  tol_distribution=ee.enum.toleranceDistribution.uniform  nSigma=4  enable_operating_limits=ee.enum.enable.no  operating_limit_action=ee.enum.passive.reportOpLim.warn  power_rating=1 W  max_working_voltage=100 V  enable_faults=ee.enum.enable.no  fault_action=simscape.enum.assert.action.none  R_faulted=inf Ohm  fault_trigger=ee.enum.faults.faultTrigger.temporal  t_fault=1 s  max_permissible_current=1 A  t_fail_on_current=1 s  noise_mode=ee.enum.sources.noise.Disabled  Tdevice=25 degC  sample_time=1e-3 s  repeatability=ee.enum.ic.repeatability.notRepeatable  user_seed=0  auto_seed=3499211588  power_derating_T1=70 degC  power_derating_T2=155 degC  operating_temperature_range_vec=[-50, 150] degC  alpha=3.93e-3 1/K  Tmeas=25 degC  thermal_mass=100 J/K  temperature_specify=off  temperature_priority=High  temperature=298.15 K  temperature_nominal_specify=off  temperature_nominal_unit=K  temperature_nominal_value=1
  Saturation : Saturate  Commented=on  UpperLimit=0.8  LowerLimit=0  ZeroCross=off
  Saturation1 : Saturate  Commented=on  UpperLimit=12  LowerLimit=0  ZeroCross=off
  Scope{,1..5,9..12} (10 alike) : Scope  Commented=on
  Scope6 : Scope
  Scope7 : Scope
  Scope8 : Scope
  Simulink-PS Converter{,1,3..4,7} (5 alike) : nesl_utility/Simulink-PS Converter  Commented=on  PhysicalDomain=network_engine_domain  SubClassName=ps_input  LeftPortType=input  RightPortType=output  PseudoPeriodic=off  Frequencies=[]  NoiseDistribution=none  NoiseParameters=[]  Unit=V  AffineConversion=on  FilteringAndDerivatives=provide  SimscapeFilterOrder=1  InputFilterTimeConstant=0.001  UdotUserProvided=0
  Simulink-PS Converter2 : nesl_utility/Simulink-PS Converter  Commented=on  PhysicalDomain=network_engine_domain  SubClassName=ps_input  LeftPortType=input  RightPortType=output  PseudoPeriodic=off  Frequencies=[]  NoiseDistribution=none  NoiseParameters=[]  Unit=1  AffineConversion=off  FilteringAndDerivatives=provide  SimscapeFilterOrder=1  InputFilterTimeConstant=0.001  UdotUserProvided=0
  Simulink-PS Converter5 : nesl_utility/Simulink-PS Converter  Commented=on  PhysicalDomain=network_engine_domain  SubClassName=ps_input  LeftPortType=input  RightPortType=output  PseudoPeriodic=off  Frequencies=[]  NoiseDistribution=none  NoiseParameters=[]  Unit=1  AffineConversion=off  FilteringAndDerivatives=provide  SimscapeFilterOrder=1  InputFilterTimeConstant=0.001  UdotUserProvided=0
  Simulink-PS Converter6 : nesl_utility/Simulink-PS Converter  PhysicalDomain=network_engine_domain  SubClassName=ps_input  LeftPortType=input  RightPortType=output  PseudoPeriodic=off  Frequencies=[]  NoiseDistribution=none  NoiseParameters=[]  Unit=V  AffineConversion=on  FilteringAndDerivatives=provide  SimscapeFilterOrder=1  InputFilterTimeConstant=0.001  UdotUserProvided=0
  Simulink-PS Converter8 : nesl_utility/Simulink-PS Converter  Commented=on  PhysicalDomain=network_engine_domain  SubClassName=ps_input  LeftPortType=input  RightPortType=output  PseudoPeriodic=off  Frequencies=[]  NoiseDistribution=none  NoiseParameters=[]  Unit=1  AffineConversion=off  FilteringAndDerivatives=provide  SimscapeFilterOrder=1  InputFilterTimeConstant=0.001  UdotUserProvided=0
  Solver Configuration{,1..3,5} (5 alike) : nesl_utility/Solver Configuration  Commented=on  PhysicalDomain=network_engine_domain  SubClassName=solver  LeftPortType=input  RightPortType=generic  Tones=[]  Harmonics=[]  SimulateNoise=off  Profile=off  UseLocalSampling=off  EnableSwitchedLinearOptims=on  FrequencyDomain=off  UseCCode=off  RelTol=0.001  AbsTol=0.001  MinStep=1e-09  ToWorkspace=off  RevertToSquareIcSolve=off  NumHomotopyIterations=100  PhasorMode=off  PhasorModeNumHarmonics=1  ConsistencySolver=NEWTON_XTOL_AFTER_FTOL  IndexReductionMethod=DerivativeReplacement  DoDC=off  ResidualTolerance=1e-09  ConsistencyTolSource=GLOBAL  ConsistencyAbsTol=0.001  ConsistencyRelTol=0.001  ConsistencyTolFactor=0.001  UseLocalSolver=off  LocalSolverChoice=NE_BACKWARD_EULER_ADVANCER  ResolveIndetEquations=on  FunctionEvalNumThread=1  LocalSolverSampleTime=0.001  DoFixedCost=off  MaxNonlinIter=3  MaxModeIter=2  ComputeImpulses=off  ImpulseIterations=2  LinearAlgebra=auto  LinearAlgebraNumThread=0  EquationFormulation=NE_TIME_EF  DelaysMemoryBudget=1024  AutomaticFiltering=on  FilteringTimeConstant=0.001  PartitionStorageMethod=AS_NEEDED  PartitionMemoryBudget=1024  PartitionMethod=ROBUST
  Solver Configuration4 : nesl_utility/Solver Configuration  PhysicalDomain=network_engine_domain  SubClassName=solver  LeftPortType=input  RightPortType=generic  Tones=[]  Harmonics=[]  SimulateNoise=off  Profile=off  UseLocalSampling=off  EnableSwitchedLinearOptims=on  FrequencyDomain=off  UseCCode=off  RelTol=0.001  AbsTol=0.001  MinStep=1e-09  ToWorkspace=off  RevertToSquareIcSolve=off  NumHomotopyIterations=100  PhasorMode=off  PhasorModeNumHarmonics=1  ConsistencySolver=NEWTON_XTOL_AFTER_FTOL  IndexReductionMethod=DerivativeReplacement  DoDC=off  ResidualTolerance=1e-09  ConsistencyTolSource=GLOBAL  ConsistencyAbsTol=0.001  ConsistencyRelTol=0.001  ConsistencyTolFactor=0.001  UseLocalSolver=off  LocalSolverChoice=NE_BACKWARD_EULER_ADVANCER  ResolveIndetEquations=on  FunctionEvalNumThread=1  LocalSolverSampleTime=0.001  DoFixedCost=off  MaxNonlinIter=3  MaxModeIter=2  ComputeImpulses=off  ImpulseIterations=2  LinearAlgebra=auto  LinearAlgebraNumThread=0  EquationFormulation=NE_TIME_EF  DelaysMemoryBudget=1024  AutomaticFiltering=on  FilteringTimeConstant=0.001  PartitionStorageMethod=AS_NEEDED  PartitionMemoryBudget=1024  PartitionMethod=ROBUST
  Step : Step  Commented=on  Time=5e-3  After=-10  SampleTime=0  ZeroCross=off
  Step1 : Step  Commented=on  Time=20e-3  After=10  SampleTime=0  ZeroCross=off
  Step_1 : Step  Commented=on  Time=4e-3  After=-1  SampleTime=0  ZeroCross=off
  Step_2 : Step  Commented=on  Time=7e-3  SampleTime=0  ZeroCross=off
  Sum : Sum  Commented=on  Inputs=|+-
  Sum1 : Sum  Commented=on  Inputs=|+++
  Sum2 : Sum  Commented=on  Inputs=|+++
  Switch_Scope : Scope  Commented=on
  Unit Delay{,1..2,4,8} (5 alike) : UnitDelay  Commented=on  SampleTime=-1  HasFrameUpgradeWarning=on
  Unit Delay3 : UnitDelay  Commented=on  SampleTime=10e-6  HasFrameUpgradeWarning=on
  Unit Delay5 : UnitDelay  Commented=on  SampleTime=10e-6  HasFrameUpgradeWarning=on
  Unit Delay6 : UnitDelay  SampleTime=-1  HasFrameUpgradeWarning=on
  Unit Delay7 : UnitDelay  SampleTime=10e-6  HasFrameUpgradeWarning=on
  Unit Delay9 : UnitDelay  Commented=on  SampleTime=10e-6  HasFrameUpgradeWarning=on
  Voltage Sensor{,1..5,9..11} (9 alike) : fl_lib/Electrical/Electrical Sensors/Voltage Sensor  Commented=on
  Voltage Sensor6 : fl_lib/Electrical/Electrical Sensors/Voltage Sensor
  Voltage Sensor7 : fl_lib/Electrical/Electrical Sensors/Voltage Sensor
  Voltage Sensor8 : fl_lib/Electrical/Electrical Sensors/Voltage Sensor
  Voltage_Scope{,1..3,5} (5 alike) : Scope  Commented=on
  Voltage_Scope4 : Scope
  duty cycle : Scope  Commented=on
  wires:
  From1/1 -> Simulink-PS Converter/1
  PS-Simulink Converter1/1 -> Goto/1, Voltage_Scope/1  "Vout"
  PS-Simulink Converter/1 -> Unit Delay1/1, Current_Scope/1  "IL"
  Ramp/1 -> Saturation1/1
  From/1 -> Sum/2
  Sum/1 -> PID Controller/1
  Repeating Sequence/1 -> Relational Operator/2
  Saturation/1 -> Unit Delay/1
  Gain/1 -> Goto1/1
  Data Type Conversion/1 -> Gain/1
  PID Controller/1 -> Saturation/1
  Unit Delay/1 -> duty cycle/1, Relational Operator/1
  PS-Simulink Converter2/1 -> Current_Scope1/1  "IL"
  PS-Simulink Converter3/1 -> Voltage_Scope1/1, Goto2/1  "Vout"
  From2/1 -> Simulink-PS Converter1/1
  Step_2/1 -> Sum1/1
  Step_1/1 -> Sum1/2
  Constant1/1 -> Sum1/3
  Sum1/1 -> Switch_Scope/1, Simulink-PS Converter2/1
  Saturation1/1 -> Sum/1
  Compare To Constant/1 -> NOT/1
  NOT/1 -> Compare/1
  Unit Delay1/1 -> Compare To Constant/1
  Relational Operator/1 -> Data Type Conversion/1
  PS-Simulink Converter5/1 -> Compare To Constant1/1, Voltage_Scope2/1, Goto3/1  "Vout"
  From4/1 -> Simulink-PS Converter3/1
  From3/1 -> PWM/4(In4)
  PWM/1(Out1) -> Goto4/1
  PS-Simulink Converter4/1 -> Current_is_greater_6A/1(In2)  "IL"
  Current_is_greater_6A/1(Out1) -> Goto5/1
  From5/1 -> PWM/3(In3)
  From7/1 -> PWM/5(In5), PWM/1(In1)
  Compare To Constant2/1 -> Scope2/1, Goto7/1  "UVLO_OK"
  PS-Simulink Converter6/1 -> Scope1/1, Unit Delay2/1
  Unit Delay2/1 -> Compare To Constant2/1
  From6/1 -> NOT2/1
  Compare To Constant1/1 -> OR/1
  OR/1 -> Unit Delay3/1
  Unit Delay3/1 -> Goto6/1, OR/2, NOT1/1
  NOT1/1 -> Scope/1  "OVP_OK"
  NOT2/1 -> PWM/2(In2)  "OVP_OK"
  NOT3/1 -> Scope3/1  "OVP_OK"
  Unit Delay5/1 -> NOT3/1, OR1/2, Goto10/1
  OR1/1 -> Unit Delay5/1
  Compare To Constant3/1 -> OR1/1
  Unit Delay4/1 -> Compare To Constant4/1
  Compare To Constant4/1 -> Goto11/1, Scope5/1  "UVLO_OK"
  Current_is_greater_6A1/1(Out1) -> Goto9/1
  PS-Simulink Converter7/1 -> Current_is_greater_6A1/1(In2)  "IL"
  From8/1 -> Simulink-PS Converter4/1
  PS-Simulink Converter8/1 -> Goto8/1, Voltage_Scope3/1, Compare To Constant3/1  "Vout"
  Constant/1 -> Sum2/1
  Step1/1 -> Sum2/2
  Step/1 -> Sum2/3
  Sum2/1 -> Scope4/1, Simulink-PS Converter5/1
  PS-Simulink Converter9/1 -> Unit Delay4/1
  OR2/1 -> Unit Delay7/1
  PS-Simulink Converter12/1 -> Unit Delay6/1
  [PWM] -> Simulink-PS Converter6/1
  [OVP_LATCH] -> NOT4/1
  NOT5/1 -> Scope6/1  "OVP_OK"
  PS-Simulink Converter10/1 -> Current_is_greater_6A2/1(In2)  "IL"
  PS-Simulink Converter11/1 -> [Vout], Voltage_Scope4/1, Compare To Constant5/1  "Vout"
  PWM1/1(Out1) -> [PWM]
  Compare To Constant6/1 -> [is_greater_20], Scope8/1  "UVLO_OK"
  Unit Delay6/1 -> Compare To Constant6/1
  Unit Delay7/1 -> NOT5/1, OR2/2, [OVP_LATCH]
  Compare To Constant5/1 -> OR2/1
  Current_is_greater_6A2/1(Out1) -> [OCP_TRIP]
  [is_greater_20] -> PWM1/5(In5), PWM1/1(In1)
  NOT4/1 -> PWM1/2(In2)  "OVP_OK"
  [Vout] -> PWM1/4(In4)
  [OCP_TRIP] -> PWM1/3(In3)
  PS-Simulink Converter13/1 -> Scope7/1  "VSW_measured"
  Compare To Constant8/1 -> Goto18/1, Scope11/1  "UVLO_OK"
  Current_is_greater_6A3/1(Out1) -> Goto21/1
  PS-Simulink Converter16/1 -> Unit Delay8/1
  From16/1 -> PWM2/5(In5), PWM2/1(In1)
  PS-Simulink Converter14/1 -> Current_is_greater_6A3/1(In2)  "IL"
  PWM2/1(Out1) -> Goto19/1
  Compare To Constant7/1 -> OR3/1
  From17/1 -> Simulink-PS Converter7/1
  OR3/1 -> Unit Delay9/1
  Unit Delay8/1 -> Compare To Constant8/1
  NOT6/1 -> PWM2/2(In2)  "OVP_OK"
  From15/1 -> NOT6/1
  PS-Simulink Converter17/1 -> Scope10/1  "VSW_measured"
  PS-Simulink Converter15/1 -> Goto20/1, Voltage_Scope5/1, Compare To Constant7/1  "Vout"
  Unit Delay9/1 -> NOT7/1, OR3/2, Goto17/1
  From14/1 -> PWM2/3(In3)
  NOT7/1 -> Scope9/1  "OVP_OK"
  From18/1 -> PWM2/4(In4)
  From Workspace/1 -> Scope12/1, Simulink-PS Converter8/1  "Vin"
  connections:
  "MOSFET (Ideal, Switching)"/RConn1 -- DC Voltage Source/LConn1 -- Solver Configuration/RConn1
  "MOSFET (Ideal, Switching)"/RConn2 -- Current Sensor/LConn1 -- Diode/RConn1
  Inductor/RConn1 -- Voltage Sensor/LConn1 -- Resistor/LConn1 -- Capacitor/LConn1
  Resistor/RConn1 -- Voltage Sensor/RConn2 -- DC Voltage Source/RConn1 -- Diode/LConn1 -- Electrical Reference/LConn1 -- Capacitor/RConn1
  Simulink-PS Converter/RConn1 -- "MOSFET (Ideal, Switching)"/LConn1
  PS-Simulink Converter/LConn1 -- Current Sensor/RConn1
  PS-Simulink Converter1/LConn1 -- Voltage Sensor/RConn1
  Inductor/LConn1 -- Current Sensor/RConn2
  "MOSFET (Ideal, Switching)1"/RConn1 -- Solver Configuration1/RConn1 -- DC Voltage Source1/LConn1
  "MOSFET (Ideal, Switching)1"/RConn2 -- Diode1/RConn1 -- Current Sensor1/LConn1
  Inductor1/RConn1 -- Capacitor1/LConn1 -- Resistor1/LConn1 -- Voltage Sensor1/LConn1
  Resistor1/RConn1 -- Capacitor1/RConn1 -- Electrical Reference1/LConn1 -- Diode1/LConn1 -- DC Voltage Source1/RConn1 -- Voltage Sensor1/RConn2
  PS-Simulink Converter2/LConn1 -- Current Sensor1/RConn1
  Inductor1/LConn1 -- Current Sensor1/RConn2
  Simulink-PS Converter1/RConn1 -- "MOSFET (Ideal, Switching)1"/LConn1
  PS-Simulink Converter3/LConn1 -- Voltage Sensor1/RConn1
  "MOSFET (Ideal, Switching)2"/RConn1 -- Voltage Sensor3/LConn1 -- Solver Configuration2/RConn1 -- DC Voltage Source2/LConn1
  "MOSFET (Ideal, Switching)2"/RConn2 -- Diode2/RConn1 -- Current Sensor2/LConn1
  Inductor2/RConn1 -- Capacitor2/LConn1 -- Resistor2/LConn1 -- Voltage Sensor2/LConn1
  Resistor2/RConn1 -- Capacitor2/RConn1 -- Electrical Reference2/LConn1 -- DC Voltage Source2/RConn1 -- Voltage Sensor3/RConn2 -- Diode2/LConn1 -- Voltage Sensor2/RConn2
  Inductor2/LConn1 -- Current Sensor2/RConn2
  PS-Simulink Converter5/LConn1 -- Voltage Sensor2/RConn1
  Simulink-PS Converter3/RConn1 -- "MOSFET (Ideal, Switching)2"/LConn1
  PS-Simulink Converter4/LConn1 -- Current Sensor2/RConn1
  PS-Simulink Converter6/LConn1 -- Voltage Sensor3/RConn1
  "MOSFET (Ideal, Switching)3"/RConn1 -- Voltage Sensor5/LConn1 -- Controlled Voltage Source/LConn1 -- Solver Configuration3/RConn1
  "MOSFET (Ideal, Switching)3"/RConn2 -- Current Sensor3/LConn1 -- Diode3/RConn1
  Inductor3/RConn1 -- Voltage Sensor4/LConn1 -- Resistor3/LConn1 -- Capacitor3/LConn1
  Resistor3/RConn1 -- Voltage Sensor4/RConn2 -- Voltage Sensor5/RConn2 -- Controlled Voltage Source/RConn2 -- Diode3/LConn1 -- Electrical Reference3/LConn1 -- Capacitor3/RConn1
  Simulink-PS Converter4/RConn1 -- "MOSFET (Ideal, Switching)3"/LConn1
  PS-Simulink Converter8/LConn1 -- Voltage Sensor4/RConn1
  Inductor3/LConn1 -- Current Sensor3/RConn2
  PS-Simulink Converter7/LConn1 -- Current Sensor3/RConn1
  Simulink-PS Converter5/RConn1 -- Controlled Voltage Source/RConn1
  Voltage Sensor5/RConn1 -- PS-Simulink Converter9/LConn1
  Voltage Sensor7/RConn2 -- DC Voltage Source3/RConn1 -- Resistor4/RConn1 -- Voltage Sensor6/RConn2 -- Capacitor4/RConn1 -- Diode4/LConn1 -- Electrical Reference4/LConn1
  Diode4/RConn1 -- Voltage Sensor8/RConn2 -- "MOSFET (Ideal, Switching)4"/RConn2 -- Current Sensor4/LConn1
  "MOSFET (Ideal, Switching)4"/RConn1 -- Voltage Sensor8/LConn1 -- DC Voltage Source3/LConn1 -- Voltage Sensor7/LConn1 -- Solver Configuration4/RConn1
  Resistor4/LConn1 -- Inductor4/RConn1 -- Capacitor4/LConn1 -- Voltage Sensor6/LConn1
  Inductor4/LConn1 -- Current Sensor4/RConn2
  Voltage Sensor7/RConn1 -- PS-Simulink Converter12/LConn1
  PS-Simulink Converter11/LConn1 -- Voltage Sensor6/RConn1
  Simulink-PS Converter6/RConn1 -- "MOSFET (Ideal, Switching)4"/LConn1
  PS-Simulink Converter10/LConn1 -- Current Sensor4/RConn1
  PS-Simulink Converter13/LConn1 -- Voltage Sensor8/RConn1
  Electrical Reference5/LConn1 -- Controlled Voltage Source1/RConn2 -- Voltage Sensor10/RConn2 -- Resistor5/RConn1 -- Voltage Sensor9/RConn2 -- Capacitor5/RConn1 -- Diode5/LConn1
  Current Sensor5/LConn1 -- Diode5/RConn1 -- Voltage Sensor11/RConn2 -- "MOSFET (Ideal, Switching)5"/RConn2
  Voltage Sensor9/LConn1 -- Resistor5/LConn1 -- Inductor5/RConn1 -- Capacitor5/LConn1
  Solver Configuration5/RConn1 -- Controlled Voltage Source1/LConn1 -- Voltage Sensor10/LConn1 -- "MOSFET (Ideal, Switching)5"/RConn1 -- Voltage Sensor11/LConn1
  Inductor5/LConn1 -- Current Sensor5/RConn2
  PS-Simulink Converter17/LConn1 -- Voltage Sensor11/RConn1
  PS-Simulink Converter14/LConn1 -- Current Sensor5/RConn1
  Voltage Sensor10/RConn1 -- PS-Simulink Converter16/LConn1
  PS-Simulink Converter15/LConn1 -- Voltage Sensor9/RConn1
  Simulink-PS Converter7/RConn1 -- "MOSFET (Ideal, Switching)5"/LConn1
  Simulink-PS Converter8/RConn1 -- Controlled Voltage Source1/RConn1
